simulink model "sm_car"  (R2025a)
settings: Solver=ode23t  StartTime=0.0  StopTime=400  MaxStep=0.4  RelTol=1e-3  AbsTol=1e-3  EnableMultiTasking=on
PreLoadFcn:
  | % Due to usability issue in Repeating Sequence block
  | warning('off','Simulink:Masking:Invalid');
  | 
  | % Eliminate unnecessary warnings in inactive variants
  | % Warnings generated only if you click through inactive variant
  | warning('off','MATLAB:nonExistentField');
  | warning('off','Simulink:Parameters:BlkParamUndefined');
PostLoadFcn:
  | set_param([bdroot '/Vehicle'],'popup_trailer','Off')
  | warning('off','sm:sli:setup:compile:LocalSolverNotSupported')
  | %sm_car_config_maneuver(bdroot,'WOT Braking');
  | sm_car_config_vehicle(bdroot,'false');
  | sm_car_config_logging(bdroot);
InitFcn:
  | sm_car_config_camera;
  | Vehicle = sm_car_vehcfg_checkConfig(Vehicle);
  | sm_car_check_tire_model(bdroot);
StartFcn:
  | tic;
StopFcn:
  | Elapsed_Sim_Time = toc;
  | % disp(['Elapsed Sim Time = ' num2str(Elapsed_Sim_Time)]);
undefined symbols (not defined in the file): Axle1D, AxleIn, Camera, Control, Driver, Free, Init, Maneuver, Pedal, RaceFix, RaceSpin, Scene, ShaftL1, ShaftL2, ShaftR1, ShaftR2, Soft, Stiff, Visual, X, xy_data_car_side, Y, Z
libraries: sm_lib x1546, nesl_utility x528, fl_lib x480, SimscapeFluids_lib x61, sdl_lib x49, simulink x29, ee_lib x7, simulink_extras x6, Linkage_Systems x4, Tire_1x2x x4, AntiRollBar_Systems x2, Linkage_Decoupled x2
(part 32 of 79)

== system sm_car/Vehicle/Vehicle/Chassis/SuspA1/Linkage Decoupled/Steer/Wheel Driven Rack 1UJoint ==
  note: System is actuated by
      | steering wheel
  In Bus Element1 : Inport  PortName=DrvBus  Element=aSteerWheel
  In Bus Element : Inport  Port=2  PortName=CtrlBus  Element=aSteerWheel
  Driver : Subsystem  Variant=on  VariantControlMode=label  LabelModeActiveChoice=None  mask{DriverHuman=DriverHuman, VariantLabel=DriverHuman.class.Value}
      mask prompts: DriverHuman "DriverHuman Data (structure)"; VariantLabel "Variant Label"
      mask init:
      | curblk = gcb;
      | 
      | % Set variant for this block 
      | set_param(curblk,'LabelModeActiveChoice',VariantLabel);
      settings: AttributesFormatString=%<LabelModeActiveChoice>
      mask Display: disp(' ')
  HPs : Subsystem
  Mux : Mux  Inputs=3
  PS-SL fRack : nesl_utility/PS-Simulink Converter  PhysicalDomain=network_engine_domain  SubClassName=ps_output  LeftPortType=input  RightPortType=output  PseudoPeriodic=off  Frequencies=[]  VectorFormat=1-D array  Unit=1  AffineConversion=off
  PS-SL xRack : nesl_utility/PS-Simulink Converter  PhysicalDomain=network_engine_domain  SubClassName=ps_output  LeftPortType=input  RightPortType=output  PseudoPeriodic=off  Frequencies=[]  VectorFormat=1-D array  Unit=1  AffineConversion=off
  PS-SL xRack1 : nesl_utility/PS-Simulink Converter  PhysicalDomain=network_engine_domain  SubClassName=ps_output  LeftPortType=input  RightPortType=output  PseudoPeriodic=off  Frequencies=[]  VectorFormat=1-D array  Unit=rad  AffineConversion=off
  PS-Simulink Converter : nesl_utility/PS-Simulink Converter  PhysicalDomain=network_engine_domain  SubClassName=ps_output  LeftPortType=input  RightPortType=output  PseudoPeriodic=off  Frequencies=[]  VectorFormat=1-D array  Unit=1  AffineConversion=off
  PS-Simulink Converter1 : nesl_utility/PS-Simulink Converter  PhysicalDomain=network_engine_domain  SubClassName=ps_output  LeftPortType=input  RightPortType=output  PseudoPeriodic=off  Frequencies=[]  VectorFormat=1-D array  Unit=1  AffineConversion=off
  PS-Simulink Converter2 : nesl_utility/PS-Simulink Converter  PhysicalDomain=network_engine_domain  SubClassName=ps_output  LeftPortType=input  RightPortType=output  PseudoPeriodic=off  Frequencies=[]  VectorFormat=1-D array  Unit=1  AffineConversion=off
  Physical Signal : nesl_utility/Simulink-PS Converter  PhysicalDomain=network_engine_domain  SubClassName=ps_input  LeftPortType=input  RightPortType=output  PseudoPeriodic=off  Frequencies=[]  NoiseDistribution=none  NoiseParameters=[]  Unit=rad  AffineConversion=off  FilteringAndDerivatives=filter  SimscapeFilterOrder=2  InputFilterTimeConstant=whl2steer_filter  UdotUserProvided=0
      settings: AttributesFormatString=|
      | Filter Time Constant
      | %<InputFilterTimeConstant> sec
  Pinion : Subsystem
  Prismatic Rack : sm_lib/Joints/Prismatic Joint  JointMode=Normal  CompositeWrenchDir=FollowerOnBase  CompositeWrenchFrame=BaseFrame  SenseConstraintForce=off  SenseConstraintTorque=off  SenseTotalForce=off  SenseTotalTorque=off  PositionTargetSpecify=on  PositionTargetPriority=High  PositionTargetValue=0  PositionTargetValueUnits=m  VelocityTargetSpecify=off  VelocityTargetPriority=High  VelocityTargetValue=0  VelocityTargetValueUnits=m/s  EquilibriumPosition=0  EquilibriumPositionUnits=m  SpringStiffness=0  SpringStiffnessUnits=N/m  DampingCoefficient=1e5*0  DampingCoefficientUnits=N/(m/s)  LowerLimitSpecify=off  LowerLimitBound=-1  LowerLimitBoundUnits=m  LowerLimitStiffness=1e6  LowerLimitStiffnessUnits=N/m  LowerLimitDamping=1e3  LowerLimitDampingUnits=N/(m/s)  LowerLimitTransitionRegionWidth=1e-4  LowerLimitTransitionRegionWidthUnits=m  UpperLimitSpecify=off  UpperLimitBound=1  UpperLimitBoundUnits=m  UpperLimitStiffness=1e6  UpperLimitStiffnessUnits=N/m  UpperLimitDamping=1e3  UpperLimitDampingUnits=N/(m/s)  UpperLimitTransitionRegionWidth=1e-4  UpperLimitTransitionRegionWidthUnits=m  TorqueActuationMode=NoTorque  MotionActuationMode=ComputedMotion  SensePosition=on  SenseVelocity=off  SenseAcceleration=off  SenseTorqueForce=on  SenseLowerLimitTorqueForce=off  SenseUpperLimitTorqueForce=off
  Rack : Subsystem  mask{hp_out=hp_out_rack, rack_mass=rack_mass, clr_rack=clr_rack, opc_rack=opc_rack, radius_rack=radius_rack}
      mask prompts: hp_out "HP Track Rod Inboard [xyz] (m)"; rack_mass "Mass (kg)"
      mask init:
      | rack_length = norm(hp_out-hp_out.*[1 -1 1]);
      mask TypeOptions rack_mass: Rack/Mass
      mask TypeOptions clr_rack: Rack/GraphicDiffuseColor
      mask TypeOptions opc_rack: Rack/GraphicOpacity
      mask TypeOptions radius_rack: Rack/CylinderRadius
      mask DialogControl cont_rack Prompt: Rack
      mask DialogControl text_rack_clr Prompt: Color [RGB]
      mask DialogControl text_rack_opc Prompt: Opac. (0-1)
      mask DialogControl text_rack_size Prompt: Size (m)
      mask DialogControl text_rack_rack Prompt: Rack
  Rack and Pinion Constraint : sm_lib/Gears and Couplings/Gears/Rack and Pinion Constraint  PinionRadius=rad_pinion  PinionRadiusUnits=m
  Ref to Pinion : Subsystem
  Ref to Rack : Subsystem
  Ref to Wheel : Subsystem
  Revolute Pinion : sm_lib/Joints/Revolute Joint  JointMode=Normal  CompositeWrenchDir=FollowerOnBase  CompositeWrenchFrame=BaseFrame  SenseConstraintForce=off  SenseConstraintTorque=off  SenseTotalForce=off  SenseTotalTorque=off  PositionTargetSpecify=off  PositionTargetPriority=High  PositionTargetValue=0  PositionTargetValueUnits=deg  VelocityTargetSpecify=off  VelocityTargetPriority=High  VelocityTargetValue=0  VelocityTargetValueUnits=deg/s  EquilibriumPosition=0  EquilibriumPositionUnits=deg  SpringStiffness=0  SpringStiffnessUnits=N*m/deg  DampingCoefficient=0  DampingCoefficientUnits=N*m/(deg/s)  LowerLimitSpecify=off  LowerLimitBound=-90  LowerLimitBoundUnits=deg  LowerLimitStiffness=1e4  LowerLimitStiffnessUnits=N*m/deg  LowerLimitDamping=10  LowerLimitDampingUnits=N*m/(deg/s)  LowerLimitTransitionRegionWidth=0.1  LowerLimitTransitionRegionWidthUnits=deg  UpperLimitSpecify=off  UpperLimitBound=90  UpperLimitBoundUnits=deg  UpperLimitStiffness=1e4  UpperLimitStiffnessUnits=N*m/deg  UpperLimitDamping=10  UpperLimitDampingUnits=N*m/(deg/s)  UpperLimitTransitionRegionWidth=0.1  UpperLimitTransitionRegionWidthUnits=deg  TorqueActuationMode=NoTorque  MotionActuationMode=ComputedMotion  SensePosition=off  SenseVelocity=off  SenseAcceleration=off  SenseTorqueForce=off  SenseLowerLimitTorqueForce=off  SenseUpperLimitTorqueForce=off
  Shaft Lower : Subsystem
  Shaft Steering : Subsystem
  Steer Mount : Subsystem
  Terminator : Terminator
  Transform Sensor : sm_lib/Frames and Transforms/Transform Sensor  MeasurementFrame=World  RotationSequence=XYX  SenseAngle=off  SenseAxis=off  SenseQ=off  SenseR=off  SenseRotationSequence=off  SenseOmegaX=off  SenseOmegaY=off  SenseOmegaZ=off  SenseOmega=off  SenseQDot=off  SenseRDot=off  SenseRotationSequenceDot=off  SenseAlphaX=off  SenseAlphaY=off  SenseAlphaZ=off  SenseAlpha=off  SenseQDDot=off  SenseRDDot=off  SenseX=on  SenseY=on  SenseZ=on  SenseXYZ=off  SenseRad=off  SenseAzim=off  SenseDist=off  SenseInc=off  SenseXDot=off  SenseYDot=off  SenseZDot=off  SenseXYZDot=off  SenseRadDot=off  SenseAzimDot=off  SenseDistDot=off  SenseIncDot=off  SenseXDDot=off  SenseYDDot=off  SenseZDDot=off  SenseXYZDDot=off  SenseRadDDot=off  SenseAzimDDot=off  SenseDistDDot=off  SenseIncDDot=off
  Universal : sm_lib/Joints/Universal Joint  JointMode=Normal  CompositeWrenchDir=FollowerOnBase  CompositeWrenchFrame=BaseFrame  SenseConstraintForce=off  SenseConstraintTorque=off  SenseTotalForce=off  SenseTotalTorque=off  RxPositionTargetSpecify=off  RxPositionTargetPriority=High  RxPositionTargetValue=0  RxPositionTargetValueUnits=deg  RxVelocityTargetSpecify=off  RxVelocityTargetPriority=High  RxVelocityTargetValue=0  RxVelocityTargetValueUnits=deg/s  RxEquilibriumPosition=0  RxEquilibriumPositionUnits=deg  RxSpringStiffness=0  RxSpringStiffnessUnits=N*m/deg  RxDampingCoefficient=0  RxDampingCoefficientUnits=N*m/(deg/s)  RxLowerLimitSpecify=off  RxLowerLimitBound=-90  RxLowerLimitBoundUnits=deg  RxLowerLimitStiffness=1e4  RxLowerLimitStiffnessUnits=N*m/deg  RxLowerLimitDamping=10  RxLowerLimitDampingUnits=N*m/(deg/s)  RxLowerLimitTransitionRegionWidth=0.1  RxLowerLimitTransitionRegionWidthUnits=deg  RxUpperLimitSpecify=off  RxUpperLimitBound=90  RxUpperLimitBoundUnits=deg  RxUpperLimitStiffness=1e4  RxUpperLimitStiffnessUnits=N*m/deg  RxUpperLimitDamping=10  RxUpperLimitDampingUnits=N*m/(deg/s)  RxUpperLimitTransitionRegionWidth=0.1  RxUpperLimitTransitionRegionWidthUnits=deg  RxTorqueActuationMode=NoTorque  RxMotionActuationMode=ComputedMotion  RxSensePosition=off  RxSenseVelocity=off  RxSenseAcceleration=off  RxSenseTorqueForce=off  RxSenseLowerLimitTorqueForce=off  RxSenseUpperLimitTorqueForce=off  RyPositionTargetSpecify=off  RyPositionTargetPriority=High  RyPositionTargetValue=0  RyPositionTargetValueUnits=deg  RyVelocityTargetSpecify=off  RyVelocityTargetPriority=High  RyVelocityTargetValue=0  RyVelocityTargetValueUnits=deg/s  RyEquilibriumPosition=0  RyEquilibriumPositionUnits=deg  RySpringStiffness=0  RySpringStiffnessUnits=N*m/deg  RyDampingCoefficient=0  RyDampingCoefficientUnits=N*m/(deg/s)  RyLowerLimitSpecify=off  RyLowerLimitBound=-90  RyLowerLimitBoundUnits=deg  RyLowerLimitStiffness=1e4  RyLowerLimitStiffnessUnits=N*m/deg  RyLowerLimitDamping=10  RyLowerLimitDampingUnits=N*m/(deg/s)  RyLowerLimitTransitionRegionWidth=0.1  RyLowerLimitTransitionRegionWidthUnits=deg  RyUpperLimitSpecify=off  RyUpperLimitBound=90  RyUpperLimitBoundUnits=deg  RyUpperLimitStiffness=1e4  RyUpperLimitStiffnessUnits=N*m/deg  RyUpperLimitDamping=10  RyUpperLimitDampingUnits=N*m/(deg/s)  RyUpperLimitTransitionRegionWidth=0.1  RyUpperLimitTransitionRegionWidthUnits=deg  RyTorqueActuationMode=NoTorque  RyMotionActuationMode=ComputedMotion  RySensePosition=off  RySenseVelocity=off  RySenseAcceleration=off  RySenseTorqueForce=off  RySenseLowerLimitTorqueForce=off  RySenseUpperLimitTorqueForce=off
  Wheel : Subsystem  Variant=on  VariantControlMode=label  LabelModeActiveChoice=FSAE  mask{VariantLabel=Wheel.class.Value}
      mask prompts: VariantLabel "Variant Label"
      mask init:
      | curblk = gcb;
      | 
      | % Set variant for this block 
      | set_param(curblk,'LabelModeActiveChoice',VariantLabel);
      mask Display: disp(' ');
  rodL : PMIOPort  Side=Right
  ref : PMIOPort  Port=2  Side=Right
  rodR : PMIOPort  Port=3  Side=Right
  Out Bus Element : Outport  VectorParamsAs1DForOutWhenUnconnected=off  PortName=meas  Element=FRack
  Out Bus Element1 : Outport  VectorParamsAs1DForOutWhenUnconnected=off  PortName=meas  Element=xRack
  Out Bus Element2 : Outport  VectorParamsAs1DForOutWhenUnconnected=off  PortName=meas  Element=aWheel
  Out Bus Element3 : Outport  VectorParamsAs1DForOutWhenUnconnected=off  PortName=meas  Element=Driver
  Out Bus Element4 : Outport  VectorParamsAs1DForOutWhenUnconnected=off  PortName=meas  Element=xyz_UJoint
  wires:
  Driver/1(m) -> Out Bus Element3/1
  In Bus Element/1 -> Physical Signal/1, Driver/1(q)
  PS-SL xRack1/1 -> Out Bus Element2/1
  In Bus Element1/1 -> Terminator/1
  PS-SL xRack/1 -> Out Bus Element1/1
  PS-SL fRack/1 -> Out Bus Element/1
  PS-Simulink Converter/1 -> Mux/1
  PS-Simulink Converter1/1 -> Mux/2
  PS-Simulink Converter2/1 -> Mux/3
  Mux/1 -> Out Bus Element4/1
  connections:
  Wheel/RConn2 -- Driver/RConn2
  Driver/RConn1 -- Wheel/RConn1
  Rack and Pinion Constraint/LConn1 -- Shaft Lower/RConn1 -- Pinion/RConn1 -- Revolute Pinion/RConn1
  rodR/RConn1 -- Rack/LConn3
  Steer Mount/RConn2 -- PS-SL xRack1/LConn1
  Shaft Steering/RConn1 -- Steer Mount/RConn1 -- Wheel/LConn1
  Shaft Lower/LConn1 -- Universal/LConn1 -- Transform Sensor/LConn1
  Shaft Steering/LConn1 -- Transform Sensor/RConn1 -- Universal/RConn1
  Ref to Rack/RConn1 -- Prismatic Rack/LConn1
  Ref to Pinion/RConn1 -- Revolute Pinion/LConn1
  PS-SL fRack/LConn1 -- Prismatic Rack/RConn3
  Rack/LConn1 -- rodL/RConn1
  HPs/LConn1 -- Ref to Pinion/LConn1 -- Ref to Wheel/LConn1 -- Ref to Rack/LConn1 -- ref/RConn1 -- Driver/LConn1
  PS-SL xRack/LConn1 -- Prismatic Rack/RConn2
  Rack and Pinion Constraint/RConn1 -- Rack/LConn2
  Physical Signal/RConn1 -- Steer Mount/LConn2
  Prismatic Rack/RConn1 -- Rack/RConn1
  Transform Sensor/RConn2 -- PS-Simulink Converter/LConn1
  Transform Sensor/RConn3 -- PS-Simulink Converter1/LConn1
  Transform Sensor/RConn4 -- PS-Simulink Converter2/LConn1
  Ref to Wheel/RConn1 -- Steer Mount/LConn1

== system sm_car/Vehicle/Vehicle/Chassis/SuspA1/Linkage Decoupled/Wheel Meas Left/Calculate Camber ==
  uvec spin axis : Inport
  Demux : Demux  Outputs=3
  Gain : Gain  Gain=-1
  Mux : Mux  Inputs=2
  Trigonometric Function1 : Trigonometry  Operator=atan2
  magnitude : Fcn  Expr=sqrt(u(1)*u(1)+u(2)*u(2))
  Camber : Outport  VectorParamsAs1DForOutWhenUnconnected=off
  wires:
  Gain/1 -> Trigonometric Function1/1
  Demux/2 -> Mux/2
  magnitude/1 -> Trigonometric Function1/2
  Mux/1 -> magnitude/1
  Demux/3 -> Gain/1
  Trigonometric Function1/1 -> Camber/1
  uvec spin axis/1 -> Demux/1
  Demux/1 -> Mux/1

== system sm_car/Vehicle/Vehicle/Chassis/SuspA1/Linkage Decoupled/Wheel Meas Left/Calculate Camber Z Axis ==
  uvec spin axis : Inport
  Demux : Demux  Outputs=3
  Mux : Mux  Inputs=2
  Trigonometric Function1 : Trigonometry  Operator=atan2
  magnitude : Fcn  Expr=sqrt(u(1)*u(1)+u(2)*u(2))
  Camber : Outport  VectorParamsAs1DForOutWhenUnconnected=off
  wires:
  Demux/1 -> Mux/1
  uvec spin axis/1 -> Demux/1
  Trigonometric Function1/1 -> Camber/1
  Demux/3 -> Trigonometric Function1/1
  Mux/1 -> magnitude/1
  magnitude/1 -> Trigonometric Function1/2
  Demux/2 -> Mux/2

== system sm_car/Vehicle/Vehicle/Chassis/SuspA1/Linkage Decoupled/Wheel Meas Left/Calculate Toe ==
  uvec spin axis : Inport
  Demux : Demux  Outputs=3
  Gain : Gain
  Gain1 : Gain
  Terminator : Terminator
  Trigonometric Function1 : Trigonometry  Operator=atan2
  Toe : Outport  VectorParamsAs1DForOutWhenUnconnected=off
  wires:
  Trigonometric Function1/1 -> Toe/1
  Gain1/1 -> Trigonometric Function1/2
  Gain/1 -> Trigonometric Function1/1
  Demux/3 -> Terminator/1
  Demux/1 -> Gain/1
  uvec spin axis/1 -> Demux/1
  Demux/2 -> Gain1/1

== system sm_car/Vehicle/Vehicle/Chassis/SuspA1/Linkage Decoupled/Wheel Meas Left/Calculate Toe X Axis ==
  uvec spin axis : Inport
  Demux : Demux  Outputs=3
  Gain : Gain
  Gain1 : Gain
  Terminator : Terminator
  Trigonometric Function1 : Trigonometry  Operator=atan2
  Toe : Outport  VectorParamsAs1DForOutWhenUnconnected=off
  wires:
  Demux/2 -> Gain1/1
  uvec spin axis/1 -> Demux/1
  Demux/1 -> Gain/1
  Demux/3 -> Terminator/1
  Gain/1 -> Trigonometric Function1/1
  Gain1/1 -> Trigonometric Function1/2
  Trigonometric Function1/1 -> Toe/1

== system sm_car/Vehicle/Vehicle/Chassis/SuspA1/Linkage Decoupled/Wheel Meas Right/Calculate Camber ==
  uvec spin axis : Inport
  Demux : Demux  Outputs=3
  Gain : Gain  Gain=-1
  Mux : Mux  Inputs=2
  Trigonometric Function1 : Trigonometry  Operator=atan2
  magnitude : Fcn  Expr=sqrt(u(1)*u(1)+u(2)*u(2))
  Camber : Outport  VectorParamsAs1DForOutWhenUnconnected=off
  wires:
  Gain/1 -> Trigonometric Function1/1
  Demux/2 -> Mux/2
  magnitude/1 -> Trigonometric Function1/2
  Mux/1 -> magnitude/1
  Demux/3 -> Gain/1
  Trigonometric Function1/1 -> Camber/1
  uvec spin axis/1 -> Demux/1
  Demux/1 -> Mux/1

== system sm_car/Vehicle/Vehicle/Chassis/SuspA1/Linkage Decoupled/Wheel Meas Right/Calculate Camber Z Axis ==
  uvec spin axis : Inport
  Demux : Demux  Outputs=3
  Mux : Mux  Inputs=2
  Trigonometric Function1 : Trigonometry  Operator=atan2
  magnitude : Fcn  Expr=sqrt(u(1)*u(1)+u(2)*u(2))
  Camber : Outport  VectorParamsAs1DForOutWhenUnconnected=off
  wires:
  Demux/1 -> Mux/1
  uvec spin axis/1 -> Demux/1
  Trigonometric Function1/1 -> Camber/1
  Demux/3 -> Trigonometric Function1/1
  Mux/1 -> magnitude/1
  magnitude/1 -> Trigonometric Function1/2
  Demux/2 -> Mux/2

== system sm_car/Vehicle/Vehicle/Chassis/SuspA1/Linkage Decoupled/Wheel Meas Right/Calculate Toe ==
  uvec spin axis : Inport
  Demux : Demux  Outputs=3
  Gain : Gain
  Gain1 : Gain
  Terminator : Terminator
  Trigonometric Function1 : Trigonometry  Operator=atan2
  Toe : Outport  VectorParamsAs1DForOutWhenUnconnected=off
  wires:
  Trigonometric Function1/1 -> Toe/1
  Gain1/1 -> Trigonometric Function1/2
  Gain/1 -> Trigonometric Function1/1
  Demux/3 -> Terminator/1
  Demux/1 -> Gain/1
  uvec spin axis/1 -> Demux/1
  Demux/2 -> Gain1/1

== system sm_car/Vehicle/Vehicle/Chassis/SuspA1/Linkage Decoupled/Wheel Meas Right/Calculate Toe X Axis ==
  uvec spin axis : Inport
  Demux : Demux  Outputs=3
  Gain : Gain
  Gain1 : Gain
  Terminator : Terminator
  Trigonometric Function1 : Trigonometry  Operator=atan2
  Toe : Outport  VectorParamsAs1DForOutWhenUnconnected=off
  wires:
  Demux/2 -> Gain1/1
  uvec spin axis/1 -> Demux/1
  Demux/1 -> Gain/1
  Demux/3 -> Terminator/1
  Gain/1 -> Trigonometric Function1/1
  Gain1/1 -> Trigonometric Function1/2
  Trigonometric Function1/1 -> Toe/1

== system sm_car/Vehicle/Vehicle/Chassis/SuspA2/Linkage/Steer/None ==
  In Bus Element1 : Inport  PortName=DrvBus  Element=aSteerWheel
  In Bus Element2 : Inport  Port=2  PortName=CtrlBus
  Body Sensor : Subsystem  mask{offset_body_sensor=Vehicle.Chassis.Body.sCG.Value}
      mask prompts: offset_body_sensor "Sensor Frame Offset [x y z] (m)"
  Constant : Constant  Value=0
  Constant1 : Constant  Value=0
  Constant2 : Constant  Value=0
  Terminator : Terminator
  Terminator1 : Terminator
  rodL : PMIOPort  Side=Right
  ref : PMIOPort  Port=2  Side=Right
  rodR : PMIOPort  Port=3  Side=Right
  Out Bus Element : Outport  VectorParamsAs1DForOutWhenUnconnected=off  PortName=meas  Element=FRack
  Out Bus Element1 : Outport  VectorParamsAs1DForOutWhenUnconnected=off  PortName=meas  Element=xRack
  Out Bus Element2 : Outport  VectorParamsAs1DForOutWhenUnconnected=off  PortName=meas  Element=aWheel
  Out Bus Element3 : Outport  VectorParamsAs1DForOutWhenUnconnected=off  PortName=meas  Element=Driver
  wires:
  In Bus Element1/1 -> Terminator/1
  Constant/1 -> Out Bus Element1/1
  Constant1/1 -> Out Bus Element/1
  In Bus Element2/1 -> Terminator1/1
  Constant2/1 -> Out Bus Element2/1
  Body Sensor/1(Body) -> Out Bus Element3/1
  connections:
  rodL/RConn1 -- Body Sensor/LConn1 -- ref/RConn1 -- rodR/RConn1

== system sm_car/Vehicle/Vehicle/Chassis/SuspA2/Linkage/Wheel Meas Left/Calculate Camber ==
  uvec spin axis : Inport
  Demux : Demux  Outputs=3
  Gain : Gain  Gain=-1
  Mux : Mux  Inputs=2
  Trigonometric Function1 : Trigonometry  Operator=atan2
  magnitude : Fcn  Expr=sqrt(u(1)*u(1)+u(2)*u(2))
  Camber : Outport  VectorParamsAs1DForOutWhenUnconnected=off
  wires:
  Gain/1 -> Trigonometric Function1/1
  Demux/2 -> Mux/2
  magnitude/1 -> Trigonometric Function1/2
  Mux/1 -> magnitude/1
  Demux/3 -> Gain/1
  Trigonometric Function1/1 -> Camber/1
  uvec spin axis/1 -> Demux/1
  Demux/1 -> Mux/1

== system sm_car/Vehicle/Vehicle/Chassis/SuspA2/Linkage/Wheel Meas Left/Calculate Camber Z Axis ==
  uvec spin axis : Inport
  Demux : Demux  Outputs=3
  Mux : Mux  Inputs=2
  Trigonometric Function1 : Trigonometry  Operator=atan2
  magnitude : Fcn  Expr=sqrt(u(1)*u(1)+u(2)*u(2))
  Camber : Outport  VectorParamsAs1DForOutWhenUnconnected=off
  wires:
  Demux/1 -> Mux/1
  uvec spin axis/1 -> Demux/1
  Trigonometric Function1/1 -> Camber/1
  Demux/3 -> Trigonometric Function1/1
  Mux/1 -> magnitude/1
  magnitude/1 -> Trigonometric Function1/2
  Demux/2 -> Mux/2

== system sm_car/Vehicle/Vehicle/Chassis/SuspA2/Linkage/Wheel Meas Left/Calculate Toe ==
  uvec spin axis : Inport
  Demux : Demux  Outputs=3
  Gain : Gain
  Gain1 : Gain
  Terminator : Terminator
  Trigonometric Function1 : Trigonometry  Operator=atan2
  Toe : Outport  VectorParamsAs1DForOutWhenUnconnected=off
  wires:
  Trigonometric Function1/1 -> Toe/1
  Gain1/1 -> Trigonometric Function1/2
  Gain/1 -> Trigonometric Function1/1
  Demux/3 -> Terminator/1
  Demux/1 -> Gain/1
  uvec spin axis/1 -> Demux/1
  Demux/2 -> Gain1/1

== system sm_car/Vehicle/Vehicle/Chassis/SuspA2/Linkage/Wheel Meas Left/Calculate Toe X Axis ==
  uvec spin axis : Inport
  Demux : Demux  Outputs=3
  Gain : Gain
  Gain1 : Gain
  Terminator : Terminator
  Trigonometric Function1 : Trigonometry  Operator=atan2
  Toe : Outport  VectorParamsAs1DForOutWhenUnconnected=off
  wires:
  Demux/2 -> Gain1/1
  uvec spin axis/1 -> Demux/1
  Demux/1 -> Gain/1
  Demux/3 -> Terminator/1
  Gain/1 -> Trigonometric Function1/1
  Gain1/1 -> Trigonometric Function1/2
  Trigonometric Function1/1 -> Toe/1

== system sm_car/Vehicle/Vehicle/Chassis/SuspA2/Linkage/Wheel Meas Right/Calculate Camber ==
  uvec spin axis : Inport
  Demux : Demux  Outputs=3
  Gain : Gain  Gain=-1
  Mux : Mux  Inputs=2
  Trigonometric Function1 : Trigonometry  Operator=atan2
  magnitude : Fcn  Expr=sqrt(u(1)*u(1)+u(2)*u(2))
  Camber : Outport  VectorParamsAs1DForOutWhenUnconnected=off
  wires:
  Gain/1 -> Trigonometric Function1/1
  Demux/2 -> Mux/2
  magnitude/1 -> Trigonometric Function1/2
  Mux/1 -> magnitude/1
  Demux/3 -> Gain/1
  Trigonometric Function1/1 -> Camber/1
  uvec spin axis/1 -> Demux/1
  Demux/1 -> Mux/1

== system sm_car/Vehicle/Vehicle/Chassis/SuspA2/Linkage/Wheel Meas Right/Calculate Camber Z Axis ==
  uvec spin axis : Inport
  Demux : Demux  Outputs=3
  Mux : Mux  Inputs=2
  Trigonometric Function1 : Trigonometry  Operator=atan2
  magnitude : Fcn  Expr=sqrt(u(1)*u(1)+u(2)*u(2))
  Camber : Outport  VectorParamsAs1DForOutWhenUnconnected=off
  wires:
  Demux/1 -> Mux/1
  uvec spin axis/1 -> Demux/1
  Trigonometric Function1/1 -> Camber/1
  Demux/3 -> Trigonometric Function1/1
  Mux/1 -> magnitude/1
  magnitude/1 -> Trigonometric Function1/2
  Demux/2 -> Mux/2

== system sm_car/Vehicle/Vehicle/Chassis/SuspA2/Linkage/Wheel Meas Right/Calculate Toe ==
  uvec spin axis : Inport
  Demux : Demux  Outputs=3
  Gain : Gain
  Gain1 : Gain
  Terminator : Terminator
  Trigonometric Function1 : Trigonometry  Operator=atan2
  Toe : Outport  VectorParamsAs1DForOutWhenUnconnected=off
  wires:
  Trigonometric Function1/1 -> Toe/1
  Gain1/1 -> Trigonometric Function1/2
  Gain/1 -> Trigonometric Function1/1
  Demux/3 -> Terminator/1
  Demux/1 -> Gain/1
  uvec spin axis/1 -> Demux/1
  Demux/2 -> Gain1/1

== system sm_car/Vehicle/Vehicle/Chassis/SuspA2/Linkage/Wheel Meas Right/Calculate Toe X Axis ==
  uvec spin axis : Inport
  Demux : Demux  Outputs=3
  Gain : Gain
  Gain1 : Gain
  Terminator : Terminator
  Trigonometric Function1 : Trigonometry  Operator=atan2
  Toe : Outport  VectorParamsAs1DForOutWhenUnconnected=off
  wires:
  Demux/2 -> Gain1/1
  uvec spin axis/1 -> Demux/1
  Demux/1 -> Gain/1
  Demux/3 -> Terminator/1
  Gain/1 -> Trigonometric Function1/1
  Gain1/1 -> Trigonometric Function1/2
  Trigonometric Function1/1 -> Toe/1

== system sm_car/Vehicle/Vehicle/Powertrain/Driveline/L1 R1 L2 R2/ShaftL1/Driveshaft Measurements ==
  Bus Creator : BusCreator  Inputs=2
  Zero : Constant  Value=0  OutDataTypeStr=Inherit: Inherit via back propagation
  Zero1 : Constant  Value=0  OutDataTypeStr=Inherit: Inherit via back propagation
  meas : Outport  VectorParamsAs1DForOutWhenUnconnected=off
  wires:
  Zero/1 -> Bus Creator/1  "w"
  Zero1/1 -> Bus Creator/2  "q"
  Bus Creator/1 -> meas/1

== system sm_car/Vehicle/Vehicle/Powertrain/Driveline/L1 R1 L2 R2/ShaftL2/Driveshaft Measurements ==
  Bus Creator : BusCreator  Inputs=2
  Zero : Constant  Value=0  OutDataTypeStr=Inherit: Inherit via back propagation
  Zero1 : Constant  Value=0  OutDataTypeStr=Inherit: Inherit via back propagation
  meas : Outport  VectorParamsAs1DForOutWhenUnconnected=off
  wires:
  Zero/1 -> Bus Creator/1  "w"
  Zero1/1 -> Bus Creator/2  "q"
  Bus Creator/1 -> meas/1

== system sm_car/Vehicle/Vehicle/Powertrain/Driveline/L1 R1 L2 R2/ShaftR1/Driveshaft Measurements ==
  Bus Creator : BusCreator  Inputs=2
  Zero : Constant  Value=0  OutDataTypeStr=Inherit: Inherit via back propagation
  Zero1 : Constant  Value=0  OutDataTypeStr=Inherit: Inherit via back propagation
  meas : Outport  VectorParamsAs1DForOutWhenUnconnected=off
  wires:
  Zero/1 -> Bus Creator/1  "w"
  Zero1/1 -> Bus Creator/2  "q"
  Bus Creator/1 -> meas/1

== system sm_car/Vehicle/Vehicle/Powertrain/Driveline/L1 R1 L2 R2/ShaftR2/Driveshaft Measurements ==
  Bus Creator : BusCreator  Inputs=2
  Zero : Constant  Value=0  OutDataTypeStr=Inherit: Inherit via back propagation
  Zero1 : Constant  Value=0  OutDataTypeStr=Inherit: Inherit via back propagation
  meas : Outport  VectorParamsAs1DForOutWhenUnconnected=off
  wires:
  Zero/1 -> Bus Creator/1  "w"
  Zero1/1 -> Bus Creator/2  "q"
  Bus Creator/1 -> meas/1

== system sm_car/Vehicle/Vehicle/Powertrain/Power/Electric L1 R1 L2 R2/Battery/Sensor VI ==
  Bus Creator : BusCreator  Inputs=2
  Current Sensor : fl_lib/Electrical/Electrical Sensors/Current Sensor
  PS-Simulink Converter2 : nesl_utility/PS-Simulink Converter  PhysicalDomain=network_engine_domain  SubClassName=ps_output  LeftPortType=input  RightPortType=output  PseudoPeriodic=off  Frequencies=[]  VectorFormat=1-D array  Unit=1  AffineConversion=off
  PS-Simulink Converter4 : nesl_utility/PS-Simulink Converter  PhysicalDomain=network_engine_domain  SubClassName=ps_output  LeftPortType=input  RightPortType=output  PseudoPeriodic=off  Frequencies=[]  VectorFormat=1-D array  Unit=1  AffineConversion=off
  Transfer Fcn1 : TransferFcn  Denominator=[.001 1]
  Transfer Fcn5 : TransferFcn  Denominator=[.001 1]
  Voltage Sensor2 : fl_lib/Electrical/Electrical Sensors/Voltage Sensor
  + : PMIOPort  Side=Left
  - : PMIOPort  Port=2  Side=Right
  G : PMIOPort  Port=3  Side=Right
  vi : Outport
  wires:
  Bus Creator/1 -> vi/1
  Transfer Fcn5/1 -> Bus Creator/1  "v"
  Transfer Fcn1/1 -> Bus Creator/2  "i"
  PS-Simulink Converter2/1 -> Transfer Fcn1/1
  PS-Simulink Converter4/1 -> Transfer Fcn5/1
  connections:
  Current Sensor/RConn1 -- PS-Simulink Converter2/LConn1
  Voltage Sensor2/RConn2 -- G/RConn1
  Current Sensor/RConn2 -- -/RConn1
  PS-Simulink Converter4/LConn1 -- Voltage Sensor2/RConn1
  Voltage Sensor2/LConn1 -- Current Sensor/LConn1 -- +/RConn1

== system sm_car/Vehicle/Vehicle/Powertrain/Power/Electric L1 R1 L2 R2/Motor L1/Sensing Current ==
  Current Sensor : fl_lib/Electrical/Electrical Sensors/Current Sensor
  PS-Simulink Converter1 : nesl_utility/PS-Simulink Converter  PhysicalDomain=network_engine_domain  SubClassName=ps_output  LeftPortType=input  RightPortType=output  PseudoPeriodic=off  Frequencies=[]  VectorFormat=1-D array  Unit=1  AffineConversion=off
  + : PMIOPort  Side=Right
  - : PMIOPort  Port=2  Side=Left
  Out1 : Outport  VectorParamsAs1DForOutWhenUnconnected=off
  wires:
  PS-Simulink Converter1/1 -> Out1/1
  connections:
  +/RConn1 -- Current Sensor/LConn1
  Current Sensor/RConn1 -- PS-Simulink Converter1/LConn1
  Current Sensor/RConn2 -- -/RConn1

== system sm_car/Vehicle/Vehicle/Powertrain/Power/Electric L1 R1 L2 R2/Motor L1/Sensing Torque ==
  Ideal Torque Sensor : fl_lib/Mechanical/Mechanical Sensors/Ideal Torque Sensor
  PS-Simulink Converter1 : nesl_utility/PS-Simulink Converter  PhysicalDomain=network_engine_domain  SubClassName=ps_output  LeftPortType=input  RightPortType=output  PseudoPeriodic=off  Frequencies=[]  VectorFormat=1-D array  Unit=1  AffineConversion=off
  R : PMIOPort  Side=Left
  C : PMIOPort  Port=2  Side=Right
  T : Outport  VectorParamsAs1DForOutWhenUnconnected=off
  wires:
  PS-Simulink Converter1/1 -> T/1
  connections:
  Ideal Torque Sensor/LConn1 -- R/RConn1
  Ideal Torque Sensor/RConn1 -- C/RConn1
  Ideal Torque Sensor/RConn2 -- PS-Simulink Converter1/LConn1

== system sm_car/Vehicle/Vehicle/Powertrain/Power/Electric L1 R1 L2 R2/Motor L2/Sensing Current ==
  Current Sensor : fl_lib/Electrical/Electrical Sensors/Current Sensor
  PS-Simulink Converter1 : nesl_utility/PS-Simulink Converter  PhysicalDomain=network_engine_domain  SubClassName=ps_output  LeftPortType=input  RightPortType=output  PseudoPeriodic=off  Frequencies=[]  VectorFormat=1-D array  Unit=1  AffineConversion=off
  + : PMIOPort  Side=Right
  - : PMIOPort  Port=2  Side=Left
  Out1 : Outport  VectorParamsAs1DForOutWhenUnconnected=off
  wires:
  PS-Simulink Converter1/1 -> Out1/1
  connections:
  +/RConn1 -- Current Sensor/LConn1
  Current Sensor/RConn1 -- PS-Simulink Converter1/LConn1
  Current Sensor/RConn2 -- -/RConn1

== system sm_car/Vehicle/Vehicle/Powertrain/Power/Electric L1 R1 L2 R2/Motor L2/Sensing Torque ==
  Ideal Torque Sensor : fl_lib/Mechanical/Mechanical Sensors/Ideal Torque Sensor
  PS-Simulink Converter1 : nesl_utility/PS-Simulink Converter  PhysicalDomain=network_engine_domain  SubClassName=ps_output  LeftPortType=input  RightPortType=output  PseudoPeriodic=off  Frequencies=[]  VectorFormat=1-D array  Unit=1  AffineConversion=off
  R : PMIOPort  Side=Left
  C : PMIOPort  Port=2  Side=Right
  T : Outport  VectorParamsAs1DForOutWhenUnconnected=off
  wires:
  PS-Simulink Converter1/1 -> T/1
  connections:
  Ideal Torque Sensor/LConn1 -- R/RConn1
  Ideal Torque Sensor/RConn1 -- C/RConn1
  Ideal Torque Sensor/RConn2 -- PS-Simulink Converter1/LConn1

== system sm_car/Vehicle/Vehicle/Powertrain/Power/Electric L1 R1 L2 R2/Motor R1/Sensing Current ==
  Current Sensor : fl_lib/Electrical/Electrical Sensors/Current Sensor
  PS-Simulink Converter1 : nesl_utility/PS-Simulink Converter  PhysicalDomain=network_engine_domain  SubClassName=ps_output  LeftPortType=input  RightPortType=output  PseudoPeriodic=off  Frequencies=[]  VectorFormat=1-D array  Unit=1  AffineConversion=off
  + : PMIOPort  Side=Right
  - : PMIOPort  Port=2  Side=Left
  Out1 : Outport  VectorParamsAs1DForOutWhenUnconnected=off
  wires:
  PS-Simulink Converter1/1 -> Out1/1
  connections:
  +/RConn1 -- Current Sensor/LConn1
  Current Sensor/RConn1 -- PS-Simulink Converter1/LConn1
  Current Sensor/RConn2 -- -/RConn1

== system sm_car/Vehicle/Vehicle/Powertrain/Power/Electric L1 R1 L2 R2/Motor R1/Sensing Torque ==
  Ideal Torque Sensor : fl_lib/Mechanical/Mechanical Sensors/Ideal Torque Sensor
  PS-Simulink Converter1 : nesl_utility/PS-Simulink Converter  PhysicalDomain=network_engine_domain  SubClassName=ps_output  LeftPortType=input  RightPortType=output  PseudoPeriodic=off  Frequencies=[]  VectorFormat=1-D array  Unit=1  AffineConversion=off
  R : PMIOPort  Side=Left
  C : PMIOPort  Port=2  Side=Right
  T : Outport  VectorParamsAs1DForOutWhenUnconnected=off
  wires:
  PS-Simulink Converter1/1 -> T/1
  connections:
  Ideal Torque Sensor/LConn1 -- R/RConn1
  Ideal Torque Sensor/RConn1 -- C/RConn1
  Ideal Torque Sensor/RConn2 -- PS-Simulink Converter1/LConn1

== system sm_car/Vehicle/Vehicle/Powertrain/Power/Electric L1 R1 L2 R2/Motor R2/Sensing Current ==
  Current Sensor : fl_lib/Electrical/Electrical Sensors/Current Sensor
  PS-Simulink Converter1 : nesl_utility/PS-Simulink Converter  PhysicalDomain=network_engine_domain  SubClassName=ps_output  LeftPortType=input  RightPortType=output  PseudoPeriodic=off  Frequencies=[]  VectorFormat=1-D array  Unit=1  AffineConversion=off
  + : PMIOPort  Side=Right
  - : PMIOPort  Port=2  Side=Left
  Out1 : Outport  VectorParamsAs1DForOutWhenUnconnected=off
  wires:
  PS-Simulink Converter1/1 -> Out1/1
  connections:
  +/RConn1 -- Current Sensor/LConn1
  Current Sensor/RConn1 -- PS-Simulink Converter1/LConn1
  Current Sensor/RConn2 -- -/RConn1

== system sm_car/Vehicle/Vehicle/Powertrain/Power/Electric L1 R1 L2 R2/Motor R2/Sensing Torque ==
  Ideal Torque Sensor : fl_lib/Mechanical/Mechanical Sensors/Ideal Torque Sensor
  PS-Simulink Converter1 : nesl_utility/PS-Simulink Converter  PhysicalDomain=network_engine_domain  SubClassName=ps_output  LeftPortType=input  RightPortType=output  PseudoPeriodic=off  Frequencies=[]  VectorFormat=1-D array  Unit=1  AffineConversion=off
  R : PMIOPort  Side=Left
  C : PMIOPort  Port=2  Side=Right
  T : Outport  VectorParamsAs1DForOutWhenUnconnected=off
  wires:
  PS-Simulink Converter1/1 -> T/1
  connections:
  Ideal Torque Sensor/LConn1 -- R/RConn1
  Ideal Torque Sensor/RConn1 -- C/RConn1
  Ideal Torque Sensor/RConn2 -- PS-Simulink Converter1/LConn1
